simulink library "Contact_Forces_Lib"  (R2024a)
settings: Solver=ode45  StartTime=0.0  StopTime=10.0  RelTol=1e-3  EnableMultiTasking=on
undefined symbols (not defined in the file or in its folder): b_contact, custom_param_1, custom_param_2, Extr_Data_Ring, k_contact, l_cone, length_cylinder, length_tube, mu_kinetic, mu_static, pen_exponent, pen_full_damp_F, rad_s_cone, radius_cylinder, radius_tube, v_thr, X, Y, Z
libraries: nesl_utility x197, sm_lib x115, $bdroot x72, simulink x20, fl_lib x4
(part 2 of 12)

== system Contact_Forces_Lib/3D ==
  Composite Forces : Subsystem
  Prototype : Subsystem
  Sphere in Sphere Force : Subsystem  mask(Sphere in Sphere Force){sphB_rad=0.3, sphF_rad=0.1, force_law=Linear, k_contact=1e4, b_contact=1e2, pen_full_damp_F=1e-4, pen_exponent=1, custom_param_1=1, custom_param_2=1, friction_law=Stick-Slip Continuous, mu_kinetic=0.5, mu_static=0.7, v_thr=0.001, vis_on=off, vis_opc_en=0, vis_clr=[0.9 0.2 0.2], vis_opc=0.7}
      mask prompts: sphB_rad "SphB, Inner Radius (m)"; sphF_rad "SphF, Outer Radius (m)"; force_law "Force Law"; k_contact "Contact Stiffness (N/m)"; b_contact "Contact Damping (N/(m/s))"; pen_full_damp_F "Penetration for full damping (m)"; pen_exponent "Penetration exponent (>=1)"; custom_param_1 "Custom Parameter 1"; custom_param_2 "Custom Parameter 2"; friction_law "Friction Law"; mu_kinetic "Coefficient of Kinetic Friction"; mu_static "Coefficient of Static Friction"; v_thr "Velocity Threshold (m/s)"; vis_on "Visualize Contact Surfaces"; vis_opc_en "Visualize Opacity Enable"; vis_clr "Color of Surface Element (RGB)"; vis_opc "Opacity of Surface Element (0-1)"
      mask help:
      | This subsystem implements a contact force between two spheres.  The force acts to keep distance from frame SphB to SphF less than (inner radius SphB - radius SphF).
      |
      | Frames connected to ports:
      | 1. Located at center of sphere
      | 2. Orientation does not matter
      |
      | Output signal is a bus with intermediate calculations and total force. Click Help for a diagram describing this force.
      mask init: same as Contact_Forces_Lib/2D/Circle to Circle Force
      mask Help: web(which('Sphere_in_Sphere_Contact.html'));
      mask TypeOptions force_law: Linear | Nonlinear | Custom
      mask Callback force_law:
      | %maskStr = get_param(gcb,'MaskValues');
      | maskObj = Simulink.Mask.get(gcb);
      | pfd_h = maskObj.getParameter('pen_full_damp_F');
      | pex_h = maskObj.getParameter('pen_exponent');
      | cc1_h = maskObj.getParameter('custom_param_1');
      | cc2_h = maskObj.getParameter('custom_param_2');
      | if strcmp(get_param(gcb,'force_law'),'Linear')
      |     pfd_h.Visible = 'off';
      |     pex_h.Visible = 'off';
      |     cc1_h.Visible = 'off';
      |     cc2_h.Visible = 'off';
      | %    set_param(gcb,'MaskVisibilities',{'on' 'on' 'on' 'on' 'on' 'off' 'off' 'off' 'off'});
      | %    set_param(gcb,'MaskVisibilities',{'on' 'on' 'on' 'on' 'on' 'off' 'off' 'off' 'off'});
      | elseif strcmp(get_param(gcb,'force_law'),'Nonlinear')
      |     pfd_h.Visible = 'on';
      |     pex_h.Visible = 'on';
      |     cc1_h.Visible = 'off';
      |     cc2_h.Visible = 'off';
      |     %set_param(gcb,'MaskVisibilities',{'on' 'on' 'on' 'on' 'on' 'on' 'on' 'off' 'off'});
      | elseif strcmp(get_param(gcb,'force_law'),'Custom')
      |     pfd_h.Visible = 'off';
      |     pex_h.Visible = 'off';
      |     cc1_h.Visible = 'on';
      |     cc2_h.Visible = 'on';
      |     %set_param(gcb,'MaskVisibilities',{'on' 'on' 'on' 'on' 'on' 'off' 'off' 'on' 'on'});
      | end
      | %clear maskObj
      | 
      | %maskObj = Simulink.Mask.get(gcb);
      | %if strcmp(get_param(gcb,'x'),'on')
      | %else
      | %    yh.Visible = 'off';
      | %end
      mask TypeOptions friction_law: None | Stick-Slip Continuous
      mask Callback friction_law:
      | maskObj = Simulink.Mask.get(gcb);
      | muk_h = maskObj.getParameter('mu_kinetic');
      | mus_h = maskObj.getParameter('mu_static');
      | vth_h = maskObj.getParameter('v_thr');
      | if strcmp(get_param(gcb,'friction_law'),'None')
      |     muk_h.Visible = 'off';
      |     mus_h.Visible = 'off';
      |     vth_h.Visible = 'off';
      | elseif strcmp(get_param(gcb,'friction_law'),'Stick-Slip Continuous')
      |     muk_h.Visible = 'on';
      |     mus_h.Visible = 'on';
      |     vth_h.Visible = 'on';
      | end
      | clear maskObj
      mask Callback vis_on:
      | maskObj = Simulink.Mask.get(gcb);
      | vis_clr_h = maskObj.getParameter('vis_clr');
      | vis_opc_h = maskObj.getParameter('vis_opc');
      | if strcmp(get_param(gcb,'vis_on'),'off')
      |     vis_clr_h.Visible = 'off';
      |     vis_opc_h.Visible = 'off';
      | elseif strcmp(get_param(gcb,'vis_on'),'on')
      |     vis_clr_h.Visible = 'on';
      |     vis_opc_h.Visible = 'on';
      | end
      | clear maskObj
      mask DialogControl Dim_Cont Prompt: Dimensions
      mask DialogControl Con_Cont Prompt: Contact
      mask DialogControl Fri_Cont Prompt: Friction
      mask DialogControl Container9 Prompt: Visual
      mask Display: image('Sphere_in_Sphere_Contact_IMAGE.jpg');
  Sphere to Cone Force : Subsystem  mask(Sphere to Cone Force){radius_sphere=1, cone_or=10, cone_ir=12, cone_theta=45, cone_h=8, active_angle=[-180 180], d_cone=0, r_cone=0, cosConeTh=0, sinConeTh=0, force_law=Linear, k_contact=1e6, b_contact=1e6, pen_full_damp_F=1e-4, pen_exponent=1, custom_param_1=1, custom_param_2=1, friction_law=Stick-Slip Continuous, mu_kinetic=0.5, mu_static=0.7, v_thr=0.001, vis_on=off, vis_opc_en=0, vis_depth_conBx=0.02, vis_clr=[0.9 0.2 0.2], vis_opc=0.7}
      mask prompts: radius_sphere "Sphere Radius (m)"; cone_or "Cone Outer Radius (m)"; cone_ir "Cone Inner Radius (m)"; cone_theta "Cone Angle (deg)"; cone_h "Cone Height (m)"; active_angle "Active Range (min, max angle (deg))"; force_law "Force Law"; k_contact "Contact Stiffness (N/m)"; b_contact "Contact Damping (N/(m/s))"; pen_full_damp_F "Penetration for full damping (m)"; pen_exponent "Penetration exponent (>=1)"; custom_param_1 "Custom Parameter 1"; custom_param_2 "Custom Parameter 2"; friction_law "Friction Law"; mu_kinetic "Coefficient of Kinetic Friction"; mu_static "Coefficient of Static Friction"; v_thr "Velocity Threshold (m/s)"; vis_on "Visualize Contact Surfaces"; vis_opc_en "Visualize Opacity Enable"; vis_depth_conBx "Radial Depth Cone Surface Elements (m)"; vis_clr "Color of Surface Element (RGB)"; vis_opc "Opacity of Surface Element (0-1)"
      mask help:
      | This subsystem implements a contact force between a sphere and a cone. The force is active outside and inside the cone.
      |
      | Frame connected to ConB port:
      | 1. Located at widest end of the cone
      | 2. Z-axis is aligned with the cone axis
      | 3. Active range: relative to +x axis of ConB [-180 180]
      |
      | Frame connected to SphF port:
      | 1. Located at center of sphere
      | 2. Orientation does not matter
      |
      | Output signal is a bus with intermediate calculations and total force. Click Help for a diagram describing this force.
      mask init:
      | d_cone = cone_or-cone_ir;
      | r_cone = (cone_or+cone_ir)/2;
      | cosConeTh = cosd(cone_theta);
      | sinConeTh = sind(cone_theta);
      | 
      | if strcmp(get_param(gcb,'force_law'),'Linear')
      |     set_param([gcb '/Forces/Force Law'],'OverrideUsingVariant','Linear');
      | elseif strcmp(get_param(gcb,'force_law'),'Nonlinear')
      |     set_param([gcb '/Forces/Force Law'],'OverrideUsingVariant','Nonlinear');
      | elseif strcmp(get_param(gcb,'force_law'),'Custom')
      |     set_param([gcb '/Forces/Force Law'],'OverrideUsingVariant','Custom');
      | end
      | 
      | if strcmp(get_param(gcb,'friction_law'),'None')
      |     set_param([gcb '/Forces/Ff/Friction Law'],'OverrideUsingVariant','None');
      | elseif strcmp(get_param(gcb,'friction_law'),'Stick-Slip Continuous')
      |     set_param([gcb '/Forces/Ff/Friction Law'],'OverrideUsingVariant','Stick_Slip_C');
      | end
      | 
      | if strcmp(get_param(gcb,'vis_on'),'on')
      |     vis_opc_en = 1;
      | elseif strcmp(get_param(gcb,'vis_on'),'off')
      |     vis_opc_en = 0;
      | end
      | 
      | frcon_xsec_in = Extr_Data_Frustum_Conical(cone_ir+vis_depth_conBx, cone_theta, cone_h, cone_ir);
      | frcon_xsec_out = Extr_Data_Frustum_Conical(cone_or, cone_theta, cone_h, cone_or-vis_depth_conBx);
      mask Help: web(which('Sphere_to_Cone_Contact.html'));
      mask TypeOptions force_law: Linear | Nonlinear | Custom
      mask Callback force_law:
      | %maskStr = get_param(gcb,'MaskValues');
      | maskObj = Simulink.Mask.get(gcb);
      | pfd_h = maskObj.getParameter('pen_full_damp_F');
      | pex_h = maskObj.getParameter('pen_exponent');
      | cc1_h = maskObj.getParameter('custom_param_1');
      | cc2_h = maskObj.getParameter('custom_param_2');
      | if strcmp(get_param(gcb,'force_law'),'Linear')
      |     pfd_h.Visible = 'off';
      |     pex_h.Visible = 'off';
      |     cc1_h.Visible = 'off';
      |     cc2_h.Visible = 'off';
      | %    set_param(gcb,'MaskVisibilities',{'on' 'on' 'on' 'on' 'on' 'off' 'off' 'off' 'off'});
      | %    set_param(gcb,'MaskVisibilities',{'on' 'on' 'on' 'on' 'on' 'off' 'off' 'off' 'off'});
      | elseif strcmp(get_param(gcb,'force_law'),'Nonlinear')
      |     pfd_h.Visible = 'on';
      |     pex_h.Visible = 'on';
      |     cc1_h.Visible = 'off';
      |     cc2_h.Visible = 'off';
      |     %set_param(gcb,'MaskVisibilities',{'on' 'on' 'on' 'on' 'on' 'on' 'on' 'off' 'off'});
      | elseif strcmp(get_param(gcb,'force_law'),'Custom')
      |     pfd_h.Visible = 'off';
      |     pex_h.Visible = 'off';
      |     cc1_h.Visible = 'on';
      |     cc2_h.Visible = 'on';
      |     %set_param(gcb,'MaskVisibilities',{'on' 'on' 'on' 'on' 'on' 'off' 'off' 'on' 'on'});
      | end
      | %clear maskObj
      | 
      | %maskObj = Simulink.Mask.get(gcb);
      | %if strcmp(get_param(gcb,'x'),'on')
      | %else
      | %    yh.Visible = 'off';
      | %end
      mask TypeOptions friction_law: None | Stick-Slip Continuous
      mask Callback friction_law:
      | maskObj = Simulink.Mask.get(gcb);
      | muk_h = maskObj.getParameter('mu_kinetic');
      | mus_h = maskObj.getParameter('mu_static');
      | vth_h = maskObj.getParameter('v_thr');
      | if strcmp(get_param(gcb,'friction_law'),'None')
      |     muk_h.Visible = 'off';
      |     mus_h.Visible = 'off';
      |     vth_h.Visible = 'off';
      | elseif strcmp(get_param(gcb,'friction_law'),'Stick-Slip Continuous')
      |     muk_h.Visible = 'on';
      |     mus_h.Visible = 'on';
      |     vth_h.Visible = 'on';
      | end
      | clear maskObj
      mask Callback vis_on:
      | maskObj = Simulink.Mask.get(gcb);
      | vis_clr_h = maskObj.getParameter('vis_clr');
      | vis_opc_h = maskObj.getParameter('vis_opc');
      | vis_depth_ConBx_h = maskObj.getParameter('vis_depth_conBx');
      | if strcmp(get_param(gcb,'vis_on'),'off')
      |     vis_depth_ConBx_h.Visible = 'off';
      |     vis_clr_h.Visible = 'off';
      |     vis_opc_h.Visible = 'off';
      | elseif strcmp(get_param(gcb,'vis_on'),'on')
      |     vis_depth_ConBx_h.Visible = 'on';
      |     vis_clr_h.Visible = 'on';
      |     vis_opc_h.Visible = 'on';
      | end
      | clear maskObj vis_clr_h vis_opc_h
      | clear vis_depth_conBx
      mask DialogControl Dim_Cont Prompt: Dimensions
      mask DialogControl Con_Cont Prompt: Contact
      mask DialogControl Fri_Cont Prompt: Friction
      mask DialogControl Vis_Cont Prompt: Visual
      mask Display: image('Sphere_to_Cone_Contact_IMAGE.jpg');
  Sphere to Plane Force : Subsystem  mask(Sphere to Plane Force){sphere_rad=0.1, plane_lenx=1, plane_leny=1, plane_depth=0.05, force_law=Linear, k_contact=1e4, b_contact=1e2, pen_full_damp_F=1e-4, pen_exponent=1, custom_param_1=1, custom_param_2=1, friction_law=Stick-Slip Continuous, mu_kinetic=0.5, mu_static=0.7, v_thr=0.001, vis_on=off, vis_opc_en=0, vis_len_plaBz=0.005, vis_clr=[0.9 0.2 0.2], vis_opc=0.7}
      mask prompts: sphere_rad "Sphere Radius (m)"; plane_lenx "Plane Length x (m)"; plane_leny "Plane Length y (m)"; plane_depth "Plane Depth to Reference Frame (m)"; force_law "Force Law"; k_contact "Contact Stiffness (N/m)"; b_contact "Contact Damping (N/(m/s))"; pen_full_damp_F "Penetration for full damping (m)"; pen_exponent "Penetration exponent (>=1)"; custom_param_1 "Custom Parameter 1"; custom_param_2 "Custom Parameter 2"; friction_law "Friction Law"; mu_kinetic "Coefficient of Kinetic Friction"; mu_static "Coefficient of Static Friction"; v_thr "Velocity Threshold (m/s)"; vis_on "Visualize Contact Surfaces"; vis_opc_en "Visualize Opacity Enable"; vis_len_plaBz "Depth Plane Surface Element (Z-Axis) (m)"; vis_clr "Color of Surface Element (RGB)"; vis_opc "Opacity of Surface Element (0-1)"
      mask help:
      | This subsystem implements a contact force between a sphere and a plane.  The force is active above and below the plane.
      |
      | Frame connected to PlaB port:
      | 1. Located at midpoint of plane (x, y, and z).
      | 2. Z-axis is normal to the surfaces where force is active.
      |
      | Frame connected to the SphF port:
      | 1. Located at center of sphere.
      | 2. Orientation does not matter.
      |
      | Output signal is a bus with intermediate calculations and total force. Click Help for a diagram describing this force.
      mask init: same as Contact_Forces_Lib/2D/Circle to Ring Force
      mask Help: web(which('Sphere_to_Plane_Contact.html'));
      mask TypeOptions force_law: Linear | Nonlinear | Custom
      mask Callback force_law:
      | %maskStr = get_param(gcb,'MaskValues');
      | maskObj = Simulink.Mask.get(gcb);
      | pfd_h = maskObj.getParameter('pen_full_damp_F');
      | pex_h = maskObj.getParameter('pen_exponent');
      | cc1_h = maskObj.getParameter('custom_param_1');
      | cc2_h = maskObj.getParameter('custom_param_2');
      | if strcmp(get_param(gcb,'force_law'),'Linear')
      |     pfd_h.Visible = 'off';
      |     pex_h.Visible = 'off';
      |     cc1_h.Visible = 'off';
      |     cc2_h.Visible = 'off';
      | %    set_param(gcb,'MaskVisibilities',{'on' 'on' 'on' 'on' 'on' 'off' 'off' 'off' 'off'});
      | %    set_param(gcb,'MaskVisibilities',{'on' 'on' 'on' 'on' 'on' 'off' 'off' 'off' 'off'});
      | elseif strcmp(get_param(gcb,'force_law'),'Nonlinear')
      |     pfd_h.Visible = 'on';
      |     pex_h.Visible = 'on';
      |     cc1_h.Visible = 'off';
      |     cc2_h.Visible = 'off';
      |     %set_param(gcb,'MaskVisibilities',{'on' 'on' 'on' 'on' 'on' 'on' 'on' 'off' 'off'});
      | elseif strcmp(get_param(gcb,'force_law'),'Custom')
      |     pfd_h.Visible = 'off';
      |     pex_h.Visible = 'off';
      |     cc1_h.Visible = 'on';
      |     cc2_h.Visible = 'on';
      |     %set_param(gcb,'MaskVisibilities',{'on' 'on' 'on' 'on' 'on' 'off' 'off' 'on' 'on'});
      | end
      | %clear maskObj
      | 
      | %maskObj = Simulink.Mask.get(gcb);
      | %if strcmp(get_param(gcb,'x'),'on')
      | %else
      | %    yh.Visible = 'off';
      | %end
      mask TypeOptions friction_law: None | Stick-Slip Continuous
      mask Callback friction_law:
      | maskObj = Simulink.Mask.get(gcb);
      | muk_h = maskObj.getParameter('mu_kinetic');
      | mus_h = maskObj.getParameter('mu_static');
      | vth_h = maskObj.getParameter('v_thr');
      | if strcmp(get_param(gcb,'friction_law'),'None')
      |     muk_h.Visible = 'off';
      |     mus_h.Visible = 'off';
      |     vth_h.Visible = 'off';
      | elseif strcmp(get_param(gcb,'friction_law'),'Stick-Slip Continuous')
      |     muk_h.Visible = 'on';
      |     mus_h.Visible = 'on';
      |     vth_h.Visible = 'on';
      | end
      | clear maskObj
      mask Callback vis_on:
      | maskObj = Simulink.Mask.get(gcb);
      | vis_clr_h = maskObj.getParameter('vis_clr');
      | vis_opc_h = maskObj.getParameter('vis_opc');
      | vis_len_plaBz_h = maskObj.getParameter('vis_len_plaBz');
      | if strcmp(get_param(gcb,'vis_on'),'off')
      |     vis_len_plaBz_h.Visible = 'off';
      |     vis_clr_h.Visible = 'off';
      |     vis_opc_h.Visible = 'off';
      | elseif strcmp(get_param(gcb,'vis_on'),'on')
      |     vis_len_plaBz_h.Visible = 'on';
      |     vis_clr_h.Visible = 'on';
      |     vis_opc_h.Visible = 'on';
      | end
      | clear maskObj vis_clr_h vis_opc_h
      | clear vis_len_plaBz_h
      mask DialogControl Dim_Cont Prompt: Dimensions
      mask DialogControl Con_Cont Prompt: Contact
      mask DialogControl Fri_Cont Prompt: Friction
      mask DialogControl Container9 Prompt: Visual
      mask Display: image('Sphere_to_Plane_Contact_IMAGE.jpg');
  Sphere to Plane Force Enabled : Subsystem  mask(Sphere to Plane Force){sphere_rad=0.1, plane_lenx=1, plane_leny=1, plane_depth=0.05, force_law=Linear, k_contact=1e4, b_contact=1e2, pen_full_damp_F=1e-4, pen_exponent=1, custom_param_1=1, custom_param_2=1, friction_law=Stick-Slip Continuous, mu_kinetic=0.5, mu_static=0.7, v_thr=0.001, vis_on=off, vis_opc_en=0, vis_len_plaBz=0.005, vis_clr=[0.9 0.2 0.2], vis_opc=0.7}
      mask prompts: sphere_rad "Sphere Radius (m)"; plane_lenx "Plane Length x (m)"; plane_leny "Plane Length y (m)"; plane_depth "Plane Depth to Reference Frame (m)"; force_law "Force Law"; k_contact "Contact Stiffness (N/m)"; b_contact "Contact Damping (N/(m/s))"; pen_full_damp_F "Penetration for full damping (m)"; pen_exponent "Penetration exponent (>=1)"; custom_param_1 "Custom Parameter 1"; custom_param_2 "Custom Parameter 2"; friction_law "Friction Law"; mu_kinetic "Coefficient of Kinetic Friction"; mu_static "Coefficient of Static Friction"; v_thr "Velocity Threshold (m/s)"; vis_on "Visualize Contact Surfaces"; vis_opc_en "Visualize Opacity Enable"; vis_len_plaBz "Depth Plane Surface Element (Z-Axis) (m)"; vis_clr "Color of Surface Element (RGB)"; vis_opc "Opacity of Surface Element (0-1)"
      mask help:
      | This subsystem implements a contact force between a sphere and a plane.  The force is active above and below the plane.
      |
      | Frame connected to PlaB port:
      | 1. Located at midpoint of plane (x, y, and z).
      | 2. Z-axis is normal to the surfaces where force is active.
      |
      | Frame connected to the SphF port:
      | 1. Located at center of sphere.
      | 2. Orientation does not matter.
      |
      | Output signal is a bus with intermediate calculations and total force. Click Help for a diagram describing this force.
      mask init: same as Contact_Forces_Lib/2D/Circle to Ring Force
      mask Help: web(which('Sphere_to_Plane_Contact.html'));
      mask TypeOptions force_law: Linear | Nonlinear | Custom
      mask Callback force_law:
      | %maskStr = get_param(gcb,'MaskValues');
      | maskObj = Simulink.Mask.get(gcb);
      | pfd_h = maskObj.getParameter('pen_full_damp_F');
      | pex_h = maskObj.getParameter('pen_exponent');
      | cc1_h = maskObj.getParameter('custom_param_1');
      | cc2_h = maskObj.getParameter('custom_param_2');
      | if strcmp(get_param(gcb,'force_law'),'Linear')
      |     pfd_h.Visible = 'off';
      |     pex_h.Visible = 'off';
      |     cc1_h.Visible = 'off';
      |     cc2_h.Visible = 'off';
      | %    set_param(gcb,'MaskVisibilities',{'on' 'on' 'on' 'on' 'on' 'off' 'off' 'off' 'off'});
      | %    set_param(gcb,'MaskVisibilities',{'on' 'on' 'on' 'on' 'on' 'off' 'off' 'off' 'off'});
      | elseif strcmp(get_param(gcb,'force_law'),'Nonlinear')
      |     pfd_h.Visible = 'on';
      |     pex_h.Visible = 'on';
      |     cc1_h.Visible = 'off';
      |     cc2_h.Visible = 'off';
      |     %set_param(gcb,'MaskVisibilities',{'on' 'on' 'on' 'on' 'on' 'on' 'on' 'off' 'off'});
      | elseif strcmp(get_param(gcb,'force_law'),'Custom')
      |     pfd_h.Visible = 'off';
      |     pex_h.Visible = 'off';
      |     cc1_h.Visible = 'on';
      |     cc2_h.Visible = 'on';
      |     %set_param(gcb,'MaskVisibilities',{'on' 'on' 'on' 'on' 'on' 'off' 'off' 'on' 'on'});
      | end
      | %clear maskObj
      | 
      | %maskObj = Simulink.Mask.get(gcb);
      | %if strcmp(get_param(gcb,'x'),'on')
      | %else
      | %    yh.Visible = 'off';
      | %end
      mask TypeOptions friction_law: None | Stick-Slip Continuous
      mask Callback friction_law:
      | maskObj = Simulink.Mask.get(gcb);
      | muk_h = maskObj.getParameter('mu_kinetic');
      | mus_h = maskObj.getParameter('mu_static');
      | vth_h = maskObj.getParameter('v_thr');
      | if strcmp(get_param(gcb,'friction_law'),'None')
      |     muk_h.Visible = 'off';
      |     mus_h.Visible = 'off';
      |     vth_h.Visible = 'off';
      | elseif strcmp(get_param(gcb,'friction_law'),'Stick-Slip Continuous')
      |     muk_h.Visible = 'on';
      |     mus_h.Visible = 'on';
      |     vth_h.Visible = 'on';
      | end
      | clear maskObj
      mask Callback vis_on:
      | maskObj = Simulink.Mask.get(gcb);
      | vis_clr_h = maskObj.getParameter('vis_clr');
      | vis_opc_h = maskObj.getParameter('vis_opc');
      | vis_len_plaBz_h = maskObj.getParameter('vis_len_plaBz');
      | if strcmp(get_param(gcb,'vis_on'),'off')
      |     vis_len_plaBz_h.Visible = 'off';
      |     vis_clr_h.Visible = 'off';
      |     vis_opc_h.Visible = 'off';
      | elseif strcmp(get_param(gcb,'vis_on'),'on')
      |     vis_len_plaBz_h.Visible = 'on';
      |     vis_clr_h.Visible = 'on';
      |     vis_opc_h.Visible = 'on';
      | end
      | clear maskObj vis_clr_h vis_opc_h
      | clear vis_len_plaBz_h
      mask DialogControl Dim_Cont Prompt: Dimensions
      mask DialogControl Con_Cont Prompt: Contact
      mask DialogControl Fri_Cont Prompt: Friction
      mask DialogControl Container9 Prompt: Visual
      mask Display: image('Sphere_to_Plane_Contact_Enabled_IMAGE.jpg');
  Sphere to Sphere Force : Subsystem  mask(Sphere to Sphere Force){sphB_rad=0.1, sphF_rad=0.1, force_law=Linear, k_contact=1e4, b_contact=1e2, pen_full_damp_F=1e-4, pen_exponent=1, custom_param_1=1, custom_param_2=1, friction_law=Stick-Slip Continuous, mu_kinetic=0.5, mu_static=0.7, v_thr=0.001, vis_on=off, vis_opc_en=0, vis_clr=[0.9 0.2 0.2], vis_opc=0.7}
      mask prompts: sphB_rad "Base Sphere Radius (SphB) (m)"; sphF_rad "Follower Sphere Radius (SphF) (m)"; force_law "Force Law"; k_contact "Contact Stiffness (N/m)"; b_contact "Contact Damping (N/(m/s))"; pen_full_damp_F "Penetration for full damping (m)"; pen_exponent "Penetration exponent (>=1)"; custom_param_1 "Custom Parameter 1"; custom_param_2 "Custom Parameter 2"; friction_law "Friction Law"; mu_kinetic "Coefficient of Kinetic Friction"; mu_static "Coefficient of Static Friction"; v_thr "Velocity Threshold (m/s)"; vis_on "Visualize Contact Surfaces"; vis_opc_en "Visualize Opacity Enable"; vis_clr "Color of Surface Element (RGB)"; vis_opc "Opacity of Surface Element (0-1)"
      mask help:
      | This subsystem implements a contact force between two spheres. It acts to repel frames SphB and SphF.
      |
      | Frames connected to ports:
      | 1. Located at center of sphere
      | 2. Orientation does not matter
      |
      | Output signal is a bus with intermediate calculations and total force. Click Help for a diagram describing this force.
      mask init: same as Contact_Forces_Lib/2D/Circle to Circle Force
      mask Help: web(which('Sphere_to_Sphere_Contact.html'));
      mask TypeOptions force_law: Linear | Nonlinear | Custom
      mask Callback force_law:
      | %maskStr = get_param(gcb,'MaskValues');
      | maskObj = Simulink.Mask.get(gcb);
      | pfd_h = maskObj.getParameter('pen_full_damp_F');
      | pex_h = maskObj.getParameter('pen_exponent');
      | cc1_h = maskObj.getParameter('custom_param_1');
      | cc2_h = maskObj.getParameter('custom_param_2');
      | if strcmp(get_param(gcb,'force_law'),'Linear')
      |     pfd_h.Visible = 'off';
      |     pex_h.Visible = 'off';
      |     cc1_h.Visible = 'off';
      |     cc2_h.Visible = 'off';
      | %    set_param(gcb,'MaskVisibilities',{'on' 'on' 'on' 'on' 'on' 'off' 'off' 'off' 'off'});
      | %    set_param(gcb,'MaskVisibilities',{'on' 'on' 'on' 'on' 'on' 'off' 'off' 'off' 'off'});
      | elseif strcmp(get_param(gcb,'force_law'),'Nonlinear')
      |     pfd_h.Visible = 'on';
      |     pex_h.Visible = 'on';
      |     cc1_h.Visible = 'off';
      |     cc2_h.Visible = 'off';
      |     %set_param(gcb,'MaskVisibilities',{'on' 'on' 'on' 'on' 'on' 'on' 'on' 'off' 'off'});
      | elseif strcmp(get_param(gcb,'force_law'),'Custom')
      |     pfd_h.Visible = 'off';
      |     pex_h.Visible = 'off';
      |     cc1_h.Visible = 'on';
      |     cc2_h.Visible = 'on';
      |     %set_param(gcb,'MaskVisibilities',{'on' 'on' 'on' 'on' 'on' 'off' 'off' 'on' 'on'});
      | end
      | %clear maskObj
      | 
      | %maskObj = Simulink.Mask.get(gcb);
      | %if strcmp(get_param(gcb,'x'),'on')
      | %else
      | %    yh.Visible = 'off';
      | %end
      mask TypeOptions friction_law: None | Stick-Slip Continuous
      mask Callback friction_law:
      | maskObj = Simulink.Mask.get(gcb);
      | muk_h = maskObj.getParameter('mu_kinetic');
      | mus_h = maskObj.getParameter('mu_static');
      | vth_h = maskObj.getParameter('v_thr');
      | if strcmp(get_param(gcb,'friction_law'),'None')
      |     muk_h.Visible = 'off';
      |     mus_h.Visible = 'off';
      |     vth_h.Visible = 'off';
      | elseif strcmp(get_param(gcb,'friction_law'),'Stick-Slip Continuous')
      |     muk_h.Visible = 'on';
      |     mus_h.Visible = 'on';
      |     vth_h.Visible = 'on';
      | end
      | clear maskObj
      mask Callback vis_on:
      | maskObj = Simulink.Mask.get(gcb);
      | vis_clr_h = maskObj.getParameter('vis_clr');
      | vis_opc_h = maskObj.getParameter('vis_opc');
      | if strcmp(get_param(gcb,'vis_on'),'off')
      |     vis_clr_h.Visible = 'off';
      |     vis_opc_h.Visible = 'off';
      | elseif strcmp(get_param(gcb,'vis_on'),'on')
      |     vis_clr_h.Visible = 'on';
      |     vis_opc_h.Visible = 'on';
      | end
      | clear maskObj
      mask DialogControl Dim_Cont Prompt: Dimensions
      mask DialogControl Con_Cont Prompt: Contact
      mask DialogControl Fri_Cont Prompt: Friction
      mask DialogControl Container13 Prompt: Visual
      mask Display: image('Sphere_to_Sphere_Contact_IMAGE.jpg');
  Sphere to Tube Force : Subsystem  mask(Sphere to Tube Force){radius_sphere=0.1, radius_tube=0.225, d_tube=0.05, l_tube=0.5, active_angle=[-180 180], force_law=Linear, k_contact=1e6, b_contact=1e5, pen_full_damp_F=1e-4, pen_exponent=1, custom_param_1=1, custom_param_2=1, friction_law=Stick-Slip Continuous, mu_kinetic=0.5, mu_static=0.7, v_thr=0.001, vis_on=off, vis_opc_en=0, vis_len_tubBx=0.225*0.02, vis_clr=[0.9 0.2 0.2], vis_opc=0.7}
      mask prompts: radius_sphere "Sphere Radius (m)"; radius_tube "Tube Radius (m)"; d_tube "Tube Thickness (m)"; l_tube "Tube Length (m)"; active_angle "Active Range (min, max angle (deg))"; force_law "Force Law"; k_contact "Contact Stiffness (N/m)"; b_contact "Contact Damping (N/(m/s))"; pen_full_damp_F "Penetration for full damping (m)"; pen_exponent "Penetration exponent (>=1)"; custom_param_1 "Custom Parameter 1"; custom_param_2 "Custom Parameter 2"; friction_law "Friction Law"; mu_kinetic "Coefficient of Kinetic Friction"; mu_static "Coefficient of Static Friction"; v_thr "Velocity Threshold (m/s)"; vis_on "Visualize Contact Surfaces"; vis_opc_en "Visualize Opacity Enable"; vis_len_tubBx "Depth Tube Surface Elements (X-Axis) (m)"; vis_clr "Color of Surface Element (RGB)"; vis_opc "Opacity of Surface Element (0-1)"
      mask help:
      | This subsystem implements a contact force between a sphere and a tube. The force is active outside and inside the tube.
      |
      | Frame connected to TubB port:
      | 1. Located at midpoint of the tube axis
      | 2. Z-axis is aligned with the tube axis
      | 3. Active range: relative to +x axis of TubB [-180 180]
      |
      | Frame connected to SphF port:
      | 1. Located at center of sphere
      | 2. Orientation does not matter
      |
      | Output signal is a bus with intermediate calculations and total force. Click Help for a diagram describing this force.
      mask init: same as Contact_Forces_Lib/2D/Circle to Ring Force
      mask Help: web(which('Sphere_to_Tube_Contact.html'));
      mask TypeOptions force_law: Linear | Nonlinear | Custom
      mask Callback force_law:
      | %maskStr = get_param(gcb,'MaskValues');
      | maskObj = Simulink.Mask.get(gcb);
      | pfd_h = maskObj.getParameter('pen_full_damp_F');
      | pex_h = maskObj.getParameter('pen_exponent');
      | cc1_h = maskObj.getParameter('custom_param_1');
      | cc2_h = maskObj.getParameter('custom_param_2');
      | if strcmp(get_param(gcb,'force_law'),'Linear')
      |     pfd_h.Visible = 'off';
      |     pex_h.Visible = 'off';
      |     cc1_h.Visible = 'off';
      |     cc2_h.Visible = 'off';
      | %    set_param(gcb,'MaskVisibilities',{'on' 'on' 'on' 'on' 'on' 'off' 'off' 'off' 'off'});
      | %    set_param(gcb,'MaskVisibilities',{'on' 'on' 'on' 'on' 'on' 'off' 'off' 'off' 'off'});
      | elseif strcmp(get_param(gcb,'force_law'),'Nonlinear')
      |     pfd_h.Visible = 'on';
      |     pex_h.Visible = 'on';
      |     cc1_h.Visible = 'off';
      |     cc2_h.Visible = 'off';
      |     %set_param(gcb,'MaskVisibilities',{'on' 'on' 'on' 'on' 'on' 'on' 'on' 'off' 'off'});
      | elseif strcmp(get_param(gcb,'force_law'),'Custom')
      |     pfd_h.Visible = 'off';
      |     pex_h.Visible = 'off';
      |     cc1_h.Visible = 'on';
      |     cc2_h.Visible = 'on';
      |     %set_param(gcb,'MaskVisibilities',{'on' 'on' 'on' 'on' 'on' 'off' 'off' 'on' 'on'});
      | end
      | %clear maskObj
      | 
      | %maskObj = Simulink.Mask.get(gcb);
      | %if strcmp(get_param(gcb,'x'),'on')
      | %else
      | %    yh.Visible = 'off';
      | %end
      mask TypeOptions friction_law: None | Stick-Slip Continuous
      mask Callback friction_law:
      | maskObj = Simulink.Mask.get(gcb);
      | muk_h = maskObj.getParameter('mu_kinetic');
      | mus_h = maskObj.getParameter('mu_static');
      | vth_h = maskObj.getParameter('v_thr');
      | if strcmp(get_param(gcb,'friction_law'),'None')
      |     muk_h.Visible = 'off';
      |     mus_h.Visible = 'off';
      |     vth_h.Visible = 'off';
      | elseif strcmp(get_param(gcb,'friction_law'),'Stick-Slip Continuous')
      |     muk_h.Visible = 'on';
      |     mus_h.Visible = 'on';
      |     vth_h.Visible = 'on';
      | end
      | clear maskObj
      mask Callback vis_on:
      | maskObj = Simulink.Mask.get(gcb);
      | vis_clr_h = maskObj.getParameter('vis_clr');
      | vis_opc_h = maskObj.getParameter('vis_opc');
      | vis_len_tubBx_h = maskObj.getParameter('vis_len_tubBx');
      | if strcmp(get_param(gcb,'vis_on'),'off')
      |     vis_len_tubBx_h.Visible = 'off';
      |     vis_clr_h.Visible = 'off';
      |     vis_opc_h.Visible = 'off';
      | elseif strcmp(get_param(gcb,'vis_on'),'on')
      |     vis_len_tubBx_h.Visible = 'on';
      |     vis_clr_h.Visible = 'on';
      |     vis_opc_h.Visible = 'on';
      | end
      | clear maskObj vis_clr_h vis_opc_h
      | clear vis_len_tubBx_h
      mask DialogControl Dim_Cont Prompt: Dimensions
      mask DialogControl Con_Cont Prompt: Contact
      mask DialogControl Fri_Cont Prompt: Friction
      mask DialogControl Vis_Cont Prompt: Visual
      mask Display: image('Sphere_to_Tube_Contact_IMAGE.jpg');
  Sphere to Tube Force Enabled : Subsystem  mask(Sphere to Tube Force){radius_sphere=0.1, radius_tube=0.225, d_tube=0.05, l_tube=0.5, active_angle=[-180 180], force_law=Linear, k_contact=1e6, b_contact=1e5, pen_full_damp_F=1e-4, pen_exponent=1, custom_param_1=1, custom_param_2=1, friction_law=Stick-Slip Continuous, mu_kinetic=0.5, mu_static=0.7, v_thr=0.001, vis_on=off, vis_opc_en=0, vis_len_tubBx=0.225*0.02, vis_clr=[0.9 0.2 0.2], vis_opc=0.7}
      mask prompts: radius_sphere "Sphere Radius (m)"; radius_tube "Tube Radius (m)"; d_tube "Tube Thickness (m)"; l_tube "Tube Length (m)"; active_angle "Active Range (min, max angle (deg))"; force_law "Force Law"; k_contact "Contact Stiffness (N/m)"; b_contact "Contact Damping (N/(m/s))"; pen_full_damp_F "Penetration for full damping (m)"; pen_exponent "Penetration exponent (>=1)"; custom_param_1 "Custom Parameter 1"; custom_param_2 "Custom Parameter 2"; friction_law "Friction Law"; mu_kinetic "Coefficient of Kinetic Friction"; mu_static "Coefficient of Static Friction"; v_thr "Velocity Threshold (m/s)"; vis_on "Visualize Contact Surfaces"; vis_opc_en "Visualize Opacity Enable"; vis_len_tubBx "Depth Tube Surface Elements (X-Axis) (m)"; vis_clr "Color of Surface Element (RGB)"; vis_opc "Opacity of Surface Element (0-1)"
      mask help:
      | This subsystem implements a contact force between a sphere and a tube. The force is active outside and inside the tube.
      |
      | Frame connected to TubB port:
      | 1. Located at midpoint of the tube axis
      | 2. Z-axis is aligned with the tube axis
      | 3. Active range: relative to +x axis of TubB [-180 180]
      |
      | Frame connected to SphF port:
      | 1. Located at center of sphere
      | 2. Orientation does not matter
      |
      | Output signal is a bus with intermediate calculations and total force. Click Help for a diagram describing this force.
      mask init: same as Contact_Forces_Lib/2D/Circle to Ring Force
      mask Help: web(which('Sphere_to_Tube_Contact.html'));
      mask TypeOptions force_law: Linear | Nonlinear | Custom
      mask Callback force_law:
      | %maskStr = get_param(gcb,'MaskValues');
      | maskObj = Simulink.Mask.get(gcb);
      | pfd_h = maskObj.getParameter('pen_full_damp_F');
      | pex_h = maskObj.getParameter('pen_exponent');
      | cc1_h = maskObj.getParameter('custom_param_1');
      | cc2_h = maskObj.getParameter('custom_param_2');
      | if strcmp(get_param(gcb,'force_law'),'Linear')
      |     pfd_h.Visible = 'off';
      |     pex_h.Visible = 'off';
      |     cc1_h.Visible = 'off';
      |     cc2_h.Visible = 'off';
      | %    set_param(gcb,'MaskVisibilities',{'on' 'on' 'on' 'on' 'on' 'off' 'off' 'off' 'off'});
      | %    set_param(gcb,'MaskVisibilities',{'on' 'on' 'on' 'on' 'on' 'off' 'off' 'off' 'off'});
      | elseif strcmp(get_param(gcb,'force_law'),'Nonlinear')
      |     pfd_h.Visible = 'on';
      |     pex_h.Visible = 'on';
      |     cc1_h.Visible = 'off';
      |     cc2_h.Visible = 'off';
      |     %set_param(gcb,'MaskVisibilities',{'on' 'on' 'on' 'on' 'on' 'on' 'on' 'off' 'off'});
      | elseif strcmp(get_param(gcb,'force_law'),'Custom')
      |     pfd_h.Visible = 'off';
      |     pex_h.Visible = 'off';
      |     cc1_h.Visible = 'on';
      |     cc2_h.Visible = 'on';
      |     %set_param(gcb,'MaskVisibilities',{'on' 'on' 'on' 'on' 'on' 'off' 'off' 'on' 'on'});
      | end
      | %clear maskObj
      | 
      | %maskObj = Simulink.Mask.get(gcb);
      | %if strcmp(get_param(gcb,'x'),'on')
      | %else
      | %    yh.Visible = 'off';
      | %end
      mask TypeOptions friction_law: None | Stick-Slip Continuous
      mask Callback friction_law:
      | maskObj = Simulink.Mask.get(gcb);
      | muk_h = maskObj.getParameter('mu_kinetic');
      | mus_h = maskObj.getParameter('mu_static');
      | vth_h = maskObj.getParameter('v_thr');
      | if strcmp(get_param(gcb,'friction_law'),'None')
      |     muk_h.Visible = 'off';
      |     mus_h.Visible = 'off';
      |     vth_h.Visible = 'off';
      | elseif strcmp(get_param(gcb,'friction_law'),'Stick-Slip Continuous')
      |     muk_h.Visible = 'on';
      |     mus_h.Visible = 'on';
      |     vth_h.Visible = 'on';
      | end
      | clear maskObj
      mask Callback vis_on:
      | maskObj = Simulink.Mask.get(gcb);
      | vis_clr_h = maskObj.getParameter('vis_clr');
      | vis_opc_h = maskObj.getParameter('vis_opc');
      | vis_len_tubBx_h = maskObj.getParameter('vis_len_tubBx');
      | if strcmp(get_param(gcb,'vis_on'),'off')
      |     vis_len_tubBx_h.Visible = 'off';
      |     vis_clr_h.Visible = 'off';
      |     vis_opc_h.Visible = 'off';
      | elseif strcmp(get_param(gcb,'vis_on'),'on')
      |     vis_len_tubBx_h.Visible = 'on';
      |     vis_clr_h.Visible = 'on';
      |     vis_opc_h.Visible = 'on';
      | end
      | clear maskObj vis_clr_h vis_opc_h
      | clear vis_len_tubBx_h
      mask DialogControl Dim_Cont Prompt: Dimensions
      mask DialogControl Con_Cont Prompt: Contact
      mask DialogControl Fri_Cont Prompt: Friction
      mask DialogControl Vis_Cont Prompt: Visual
      mask Display: image('Sphere_to_Tube_Contact_Enabled_IMAGE.jpg');

== system Contact_Forces_Lib/Constraints ==
  Cam Roller Constraint : Subsystem  mask(Cam Roller Constraint){cam_xc=[0.05*cosd(0:1:359); 0.03*sind(0:1:359)]', roller_side=Outside, cam_extr_data=[0.05*cosd(0:1:360) 0.005*cosd(360:-1:0); 0.03*sind(0:1:360) 0.005*sind(360:-1:0)]', cam_thk=0.01, cam_rho=1000, roller_curve=0, cam_clr=[0.2 0.4 0.6], cam_opc=1, roller_curve_clr=[1 1 1]*0.5, roller_curve_opc=0, roller_rad=0.02, roller_thk=0.01, roller_rho=1000, roller_clr=[1 1 1]*0.8, roller_opc=1}
      mask prompts: cam_xc "Cam Profile [x y] (m)"; roller_side "Roller Placement on Profile"; cam_extr_data "Cam Extrusion [x y] (m)"; cam_thk "Thickness (m)"; cam_rho "Density (kg/m^3)"; roller_curve "Cam Roller Curve [x y] (m)"; cam_clr "Color [RGB]"; cam_opc "Opacity (0-1)"; roller_curve_clr "Color [RGB]"; roller_curve_opc "Opacity (0-1)"; roller_rad "Radius (m)"; roller_thk "Thickness (m)"; roller_rho "Density (kg/m^3)"; roller_clr "Color [RGB]"; roller_opc "Opacity (0-1)"
      mask help: Models cam and a circular roller constrained to one another by a Point on Curve Constraint. The spline is calculated based on the cam exterior profile and the roller radius. The radius of any concave segments of the cam profile must be larger than the radius of the roller.
      mask init:
      | roller_curve = Extr_Data_Cam_Roller_Curve(cam_xc,roller_rad,get_param(gcb,'roller_side'));
      mask TypeOptions roller_side: Outside | Inside
      mask DialogControl cont_cam Prompt: Cam
      mask DialogControl push_plotcurve Prompt: Plot Cam and Roller Curve
      mask DialogControl push_plotcurve Callback:
      | v = get_param(gcb,'MaskWSVariables');
      | getMaskValue = containers.Map({v.Name}',{v.Value}');
      | assignin('base','cam_xc',getMaskValue('cam_xc'));
      | assignin('base','roller_rad',getMaskValue('roller_rad'));
      | if(getMaskValue('roller_side')==2)
      |     assignin('base','inout','Inside');
      | else
      |     assignin('base','inout','Outside');
      | end
      | evalin('base',...
      |     sprintf('Extr_Data_Cam_Roller_Curve(cam_xc,roller_rad,inout,''plot'');'));
      mask DialogControl cont_cam_vis Prompt: Cam Visualization
      mask DialogControl cont_roller_curve_vis Prompt: Roller Curve Visualization
      mask DialogControl cont_roller Prompt: Roller
      mask DialogControl cont_roller_vis Prompt: Visualization
      mask Display:
      | patch(cam_extr_data(:,1)',cam_extr_data(:,2)',[0.2 0.4 0.6]);
      | color('white')
      | plot(min(cam_extr_data(:,1))*3*0.7,min(cam_extr_data(:,2))*2*0.7);
      | plot(max(cam_extr_data(:,1))*3*0.7,max(cam_extr_data(:,2))*2*0.7);

== system Contact_Forces_Lib/Force Law ==
  note: 1) Only subsystems can be added as variant choices at this level
      | 2) Blocks cannot be connected at this level as connectivity is
      | automatically determined at simulation, based on the active variant
  Pen : Inport
  Pen Vel : Inport  Port=2
  Custom : Subsystem  VariantControl=Custom  mask(Custom Force Law){k_pen=k_contact, b_penvel=b_contact, cust_param_1=custom_param_1, cust_param_2=custom_param_2}
      mask prompts: k_pen "Contact Stiffness"; b_penvel "Contact Damping"; cust_param_1 "Custom Parameter 1"; cust_param_2 "Custom Parameter 2"
      mask help: This subsystem is for prototyping a custom force law. You can create your own force law in this subsystem and use it in the contact force models in this library by selecting the "Custom" option for the Force Law parameter.
  Linear : Subsystem  VariantControl=Linear  mask(Linear Force Law){k_pen=k_contact, b_penvel=b_contact}
      mask prompts: k_pen "Contact Stiffness"; b_penvel "Contact Damping"
      mask help: Implements a contact force law as a linear spring damper. The damping force is applied only as the penetration depth increases.
      mask Help: web(which('Force_Laws.html'));
  Nonlinear : Subsystem  VariantControl=Nonlinear  mask(Nonlinear Force Law){k_pen=k_contact, b_penvel=b_contact, pen_full_damping=pen_full_damp_F, pen_exp=pen_exponent}
      mask prompts: k_pen "Contact Stiffness"; b_penvel "Contact Damping"; pen_full_damping "Penetration for Full Damping"; pen_exp "Penetration Exponent (>=1)"
      mask help: Implements a contact force law as a nonlinear spring damper. The spring force increases exponentially with penetration. The damping force is multiplied by a scaling factor which is dependent upon the penetration. The scaling factor increases from 0 to 1 as a smooth polynomial until the penetration reaches the value specified by the parameter Penetration for Full Damping. The damping force is applied only as the penetration depth increases.
      mask Help: web(which('Force_Laws.html'));
  Spr F : Outport  VectorParamsAs1DForOutWhenUnconnected=off
  Damp F : Outport  Port=2  VectorParamsAs1DForOutWhenUnconnected=off

== system Contact_Forces_Lib/Friction Law ==
  note: 1) Only subsystems can be added as variant choices at this level
      | 2) Blocks cannot be connected at this level as connectivity is
      | automatically determined at simulation, based on the active variant
  Fn : Inport
  v : Inport  Port=2
  None : Subsystem  VariantControl=None  mask(No Friction){}
      mask help: Friction Force = 0
  "Stick-Slip C " : Subsystem  VariantControl=Stick_Slip_C  mask(Stick-Slip Friction, Continuous){muk=mu_kinetic, mus=mu_static, vth=v_thr}
      mask prompts: muk "Coefficient of Kinetic Friction"; mus "Coefficient of Static Friction"; vth "Velocity Threshold"
      mask help: Implements a continuous stick-slip friction model. Smaller velocity threshold is closer to reality but results in a numerically stiffer system.
  Ff : Outport  VectorParamsAs1DForOutWhenUnconnected=off

== system Contact_Forces_Lib/Friction Utilities ==
  Stick-Slip Friction 1D : Subsystem  mask(Stick-Slip Friction){fn_axis=Use Value, mu_kinetic=0.5, mu_static=0.8, vel_th=0.01, filt_const=1e-2}
      mask prompts: fn_axis "Normal Force (Fc Input):"; mu_kinetic "Coefficient of Kinetic Friction"; mu_static "Coefficient of Static Friction"; vel_th "Velocity Threshold"; filt_const "Low Pass Filter Constant"
      mask help:
      | Implements Stick-Slip Friction on a Simscape Multibody Joint.
      |
      | Connect the Constraint Force Output of the Simscape Multibody Joint to the Fc input and select the axis of the normal force from the parameter below.  If the model provides the Normal Force directly (Fc input is not a 3x1 vector) select "Use Value".
      |
      | Connect the velocity output from the Simscape Multibody joint to the v input.
      |
      | Lower values for Velocity Threshold and Low Pass Filter Constant makes the model closer to reality but result in a numerically stiffer system.
      mask init:
      | maskStr = get_param(gcb,'MaskValues');
      | if strcmp(maskStr{1}(1),'X')
      |     set_param([gcb '/Product'],'OverrideUsingVariant','FcVect');
      |     set_param([gcb '/Selector'],'Indices','[1]');
      | elseif strcmp(maskStr{1}(1),'Y')
      |     set_param([gcb '/Product'],'OverrideUsingVariant','FcVect');
      |     set_param([gcb '/Selector'],'Indices','[2]');
      | elseif strcmp(maskStr{1}(1),'Z')
      |     set_param([gcb '/Product'],'OverrideUsingVariant','FcVect');
      |     set_param([gcb '/Selector'],'Indices','[3]');
      | elseif strcmp(maskStr{1}(1),'U')
      |     set_param([gcb '/Product'],'OverrideUsingVariant','FcConst');
      | end
      | clear MaskStr;
      mask TypeOptions fn_axis: X-Axis | Y-Axis | Z-Axis | Use Value
  Utilities : Subsystem

== system Contact_Forces_Lib/Math ==
  Cross Product : Subsystem

== system Contact_Forces_Lib/Other Forces ==
  Attraction Force : Subsystem  mask(Attraction Force Law){k_pen=-1e5, b_penvel=10, max_sep=0.01, deadzone=0.6667}
      mask prompts: k_pen "Attraction Stiffness"; b_penvel "Attraction Damping"; max_sep "Maximum Separation"
      mask help: Implements a contact force law as a linear spring damper. The force acts to pull the two frames together.

== system Contact_Forces_Lib/2D/Circle to Circle Force ==
  Bus Creator : BusCreator  Inputs=7
  Bus Creator1 : BusCreator  Inputs=3
  Calculate Penetration : Subsystem
  External Force and Torque CirB : sm_lib/Forces and Torques/External Force and Torque  EnableForceX=on  EnableForceY=on  EnableForceZ=off  EnableForce=off  ForceResolutionFrame=AttachedFrame  EnableTorqueX=off  EnableTorqueY=off  EnableTorqueZ=on  EnableTorque=off  TorqueResolutionFrame=AttachedFrame
  External Force and Torque CirF : sm_lib/Forces and Torques/External Force and Torque  EnableForceX=on  EnableForceY=on  EnableForceZ=off  EnableForce=off  ForceResolutionFrame=AttachedFrame  EnableTorqueX=off  EnableTorqueY=off  EnableTorqueZ=on  EnableTorque=off  TorqueResolutionFrame=AttachedFrame
  Ff : Subsystem
  Fn : Subsystem
  Force Law : $bdroot/Force Law  SystemSampleTime=-1  LabelModeActiveChoice=Linear  VariantActivationTime=update diagram  AllowFlexibleInterface=on  Latency=0  AutoFrameSizeCalculation=off
  Interval Test : simulink/Logic and Bit Operations/Interval Test  IntervalClosedRight=on  uplimit=active_angle(2)  IntervalClosedLeft=on  lowlimit=active_angle(1)  OutDataTypeStr=uint8
  Product1 : Product
  Sensing : Subsystem
  Sum : Subsystem
  Sum1 : Sum  Inputs=+-
  Visual CirB : sm_lib/Body Elements/Extruded Solid  ExtrusionType=General  PolygonNumSides=3  PolygonOuterRadius=1  PolygonOuterRadiusUnits=m  ExportEntireGeometry=off  ExtrusionCrossSection=Extr_Data_Ring(cirB_rad,cirB_rad-vis_len_cirBx,active_angle(1),active_angle(2))  ExtrusionCrossSectionUnits=m  ExportConvexHullGeometry=off  ExtrusionLength=vis_len_cirBz  ExtrusionLengthUnits=m  InertiaType=CalculateFromGeometry  BasedOnType=Density  Density=0  DensityUnits=kg/(m^3)  Mass=1  MassUnits=kg  CenterOfMass=[0 0 0]  CenterOfMassUnits=m  MomentsOfInertia=[1 1 1]  MomentsOfInertiaUnits=kg*m^2  ProductsOfInertia=[0 0 0]  ProductsOfInertiaUnits=kg*m^2  GraphicType=FromGeometry  MarkerShape=Sphere  MarkerSize=10  GraphicVisPropType=SimpleVisualProperties  GraphicDiffuseColor=vis_clr  GraphicOpacity=vis_opc*vis_opc_en  GraphicSpecularColor=[0.5 0.5 0.5 1.0]  GraphicAmbientColor=[0.15 0.15 0.15 1.0]  GraphicEmissiveColor=[0.0 0.0 0.0 1.0]  GraphicShininess=75  DoExposeReferenceFrame=on  SerializedFrames=<Frames/>
  Visual CirF : sm_lib/Body Elements/Extruded Solid  ExtrusionType=General  PolygonNumSides=3  PolygonOuterRadius=1  PolygonOuterRadiusUnits=m  ExportEntireGeometry=off  ExtrusionCrossSection=Extr_Data_Ring(cirF_rad,cirF_rad-vis_len_cirFx,0,360)  ExtrusionCrossSectionUnits=m  ExportConvexHullGeometry=off  ExtrusionLength=vis_len_cirFz  ExtrusionLengthUnits=m  InertiaType=CalculateFromGeometry  BasedOnType=Density  Density=0  DensityUnits=kg/(m^3)  Mass=1  MassUnits=kg  CenterOfMass=[0 0 0]  CenterOfMassUnits=m  MomentsOfInertia=[1 1 1]  MomentsOfInertiaUnits=kg*m^2  ProductsOfInertia=[0 0 0]  ProductsOfInertiaUnits=kg*m^2  GraphicType=FromGeometry  MarkerShape=Sphere  MarkerSize=10  GraphicVisPropType=SimpleVisualProperties  GraphicDiffuseColor=vis_clr  GraphicOpacity=vis_opc*vis_opc_en  GraphicSpecularColor=[0.5 0.5 0.5 1.0]  GraphicAmbientColor=[0.15 0.15 0.15 1.0]  GraphicEmissiveColor=[0.0 0.0 0.0 1.0]  GraphicShininess=75  DoExposeReferenceFrame=on  SerializedFrames=<Frames/>
  CirF : PMIOPort  Tag=PMCPort  Side=Left
  CirB : PMIOPort  Tag=PMCPort  Port=2  Side=Right
  Out : Outport  VectorParamsAs1DForOutWhenUnconnected=off
  wires:
  Ff/6(TzCirB) -> Sum/10(TzCirB)
  Ff/5(TzCirF) -> Sum/9(TzCirF)
  Ff/4(FyCirB) -> Sum/8(FfyCirB)
  Ff/3(FxCirB) -> Sum/7(FfxCirB)
  Ff/2(FyCirF) -> Sum/6(FfyCirF)
  Ff/1(FxCirF) -> Sum/5(FfxCirF)
  Fn/4(FyCirB) -> Sum/4(FnyCirB)
  Fn/3(FxCirB) -> Sum/3(FnxCirB)
  Fn/2(FyCirF) -> Sum/2(FnyCirF)
  Fn/1(FxCirF) -> Sum/1(FnxCirF)
  Calculate Penetration/1(Pen) -> Bus Creator/2, Force Law/1, Ff/3(Pen)  "Penetration"
  Force Law/1 -> Sum1/1, Bus Creator/5  "Spr Force"
  Sensing/1(rad) -> Bus Creator1/1, Calculate Penetration/1(rad), Ff/4(rad)  "rad"
  Force Law/2 -> Bus Creator/4, Sum1/2  "Damp Force"
  Sensing/2(vrad) -> Bus Creator1/2, Calculate Penetration/2(vrad)  "vrad"
  Calculate Penetration/2(Pen Vel) -> Bus Creator/3, Force Law/2  "Penetration Vel"
  Product1/1 -> Fn/1(Fn), Bus Creator/6, Ff/1(Fn)  "Normal Force"
  Sensing/3(azm) -> Interval Test/1, Fn/3(azm), Ff/2(azm), Bus Creator1/3  "azm"
  Bus Creator/1 -> Out/1
  Bus Creator1/1 -> Bus Creator/1  "Frame Sep"
  Interval Test/1 -> Product1/2
  Sum1/1 -> Product1/1
  Sensing/4(R) -> Fn/2(R), Ff/5(R)
  Ff/7(Ff) -> Bus Creator/7  "Friction Force"
  Sensing/5(wz) -> Ff/6(wz)
  Sensing/6(vazm) -> Ff/7(vazm)
  connections:
  Sum/RConn6 -- External Force and Torque CirB/LConn3
  Sum/RConn5 -- External Force and Torque CirB/LConn2
  Sum/RConn4 -- External Force and Torque CirB/LConn1
  Sum/RConn3 -- External Force and Torque CirF/LConn3
  Sum/RConn2 -- External Force and Torque CirF/LConn2
  Sum/RConn1 -- External Force and Torque CirF/LConn1
  CirB/RConn1 -- Sensing/LConn2 -- External Force and Torque CirB/RConn1 -- Visual CirB/RConn1
  CirF/RConn1 -- External Force and Torque CirF/RConn1 -- Visual CirF/RConn1 -- Sensing/LConn1
